simulink model "pmsm"  (R2025a)
settings: Solver=FixedStepAuto  StartTime=0.0  StopTime=5  RelTol=1e-3
model workspace (MAT data in the model file):
  pmsm_Ts = Simulink.Parameter
  pmsm_Ts.Value = 1e-05
  pmsm_Ts.Complexity = 'real'
  pmsm_Ts.Dimensions = [1 1]
  pmsm_Ts.DataType = 'auto'
  pmsm_Ts.DocUnits = 's'
  pmsm_Vcc = Simulink.Parameter
  pmsm_Vcc.Value = 40
  pmsm_Vcc.Complexity = 'real'
  pmsm_Vcc.Dimensions = [1 1]
  pmsm_Vcc.DataType = 'auto'
  pmsm_Vcc.DocUnits = 'V'
  pole_pairs = Simulink.Parameter
  pole_pairs.Value = 7
  pole_pairs.Complexity = 'real'
  pole_pairs.Dimensions = [1 1]
  pole_pairs.DataType = 'auto'
libraries: nesl_utility x5, fl_lib x4, ee_lib x3, simulink_extras x3, sdl_lib x1
settings Model: Creator=ascalzo  LastModifiedBy=mfussi
settings SolverCC: EnableFixedStepZeroCrossing=on
settings DataIOCC: SaveOutput=off  DSMLogging=off  SaveTime=off
settings DebuggingCC: ParameterPrecisionLossMsg=none  UnconnectedInputMsg=warning  UnconnectedOutputMsg=warning  UnconnectedLineMsg=warning
settings ModelReferenceCC: EnableRefExpFcnMdlSchedulingChecks=on
settings RTWCC: GPUComputeCapability=3.5  DLArmComputeVersion=19.05

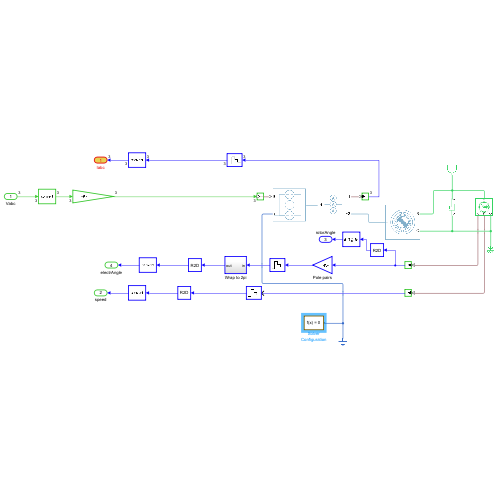
[thumbnail: Simulink's stored preview of the top-level diagram]
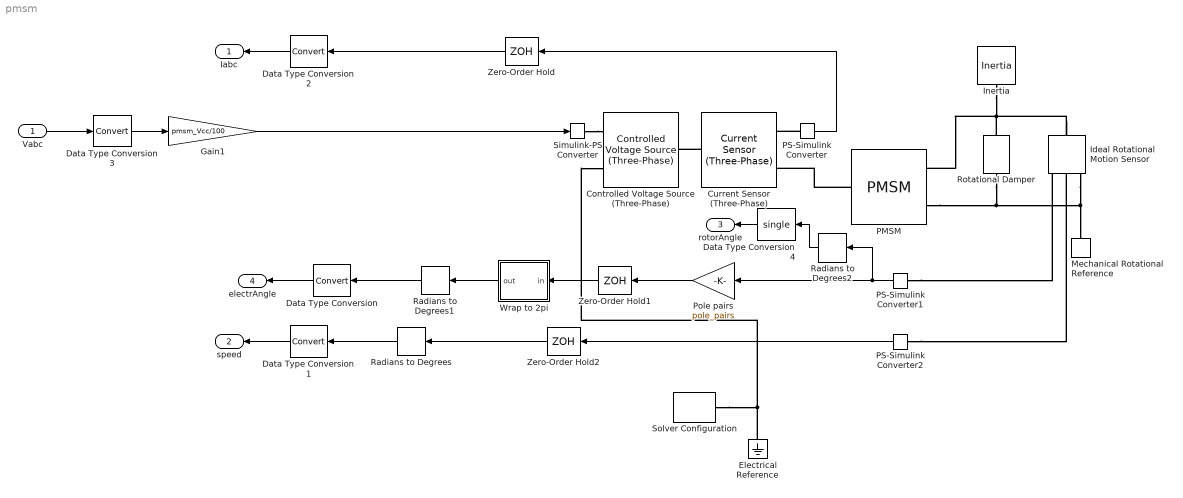
== system pmsm ==
  Vabc : Inport  OutDataTypeStr=single  Unit=%  PortDimensions=3  SampleTime=pmsm_Ts
  Controlled Voltage Source (Three-Phase) : ee_lib/Sources/Controlled Voltage Source (Three-Phase)  input_option=ee.enum.inputType.instantaneous  FRated=60 Hz
      settings: InternalSimscapePortConfiguration="{\"Bottom\":[],\"Left\":[{\"id\":\"S\",\"label\":\"S\",\"type\":\"input\"},{\"id\":\"n\",\"label\":\"n\",\"type\":\"foundation.electrical.electrical\"}],\"Right\":[{\"id\":\"N\",\"label\":\"~\",\"type\":\"foundation.electrical.three_phase\"}],\"Top\":[]}"
  Current Sensor (Three-Phase) : ee_lib/Sensors & Transducers/Current Sensor (Three-Phase)
  Data Type Conversion{,1..3} (4 alike) : DataTypeConversion  SaturateOnIntegerOverflow=off  RndMeth=Floor
  Data Type Conversion4 : DataTypeConversion  OutDataTypeStr=single  SaturateOnIntegerOverflow=off  RndMeth=Floor
  Electrical Reference : fl_lib/Electrical/Electrical Elements/Electrical Reference
  Gain1 : Gain  Gain=pmsm_Vcc/100
  Ideal Rotational Motion Sensor : fl_lib/Mechanical/Mechanical Sensors/Ideal Rotational Motion Sensor  reference=foundation.enum.MeasurementReference.difference  acceleration_port=false  velocity_port=true  position_port=true  wrap_angle=false  offset=0 rad
  Inertia : fl_lib/Mechanical/Rotational Elements/Inertia  inertia=3 g*cm^2  num_ports=foundation.enum.numPorts2.one  w_specify=off  w_priority=High  w=0 rad/s  w_nominal_specify=off  w_nominal_value=1  w_nominal_unit=rad/s  t_specify=off  t_priority=None  t=0 N*m  t_nominal_specify=off  t_nominal_value=1  t_nominal_unit=N*m
  Mechanical Rotational Reference : fl_lib/Mechanical/Rotational Elements/Mechanical Rotational Reference
  PMSM : ee_lib/Electromechanical/Permanent Magnet/PMSM  port_option=ee.enum.threePhasePort.composite  winding_type=ee.enum.statorconnection.wye  machine_param=ee.enum.pmsm.parameterization.constant  nPolePairs=pole_pairs  pmflux_param=ee.enum.pmflux.torqueconstant  pm_flux_linkage=0.03 Wb  torque_constant=32.2*2/3 mN*m/A  back_emf_constant=0.18 V/(rad/s)  stator_param=ee.enum.statorparam.LsLmMs  Ld=0.00019 H  Lq=0.00025 H  idVec=[-200, 0, 200] A  iqVec=[-200, 0, 200] A  LdMatrix=0.0002 * ones(3, 3) H  LqMatrix=0.0002 * ones(3, 3) H  PmMatrix=0.1 * ones(3, 3) Wb  ktMatrix=0.18 * ones(3, 3) N*m/A  keMatrix=0.18 * ones(3, 3) V/(rad/s)  L0=0.00016 H  Ls=3150/3 uH  Lm=-0.1*3150/3*0 uH  Ms=(3150/3)/2 uH  Rs=0.9 % 25.9/2 Ohm  zero_sequence=ee.enum.park.zerosequence.exclude  axes_param=ee.enum.rotorangle.daxis  loss_param=ee.enum.ironloss.none  losses_oc=[0, 0, 0] W  losses_sc=[0, 0, 0] W  f_losses=60 Hz  Isc_losses=95 A  J=3.3 g*cm^2  lam=7.4e-5 m*mN/rpm  i_d_specify=off  i_d_priority=None  i_d=0 A  i_d_nominal_specify=off  i_d_nominal_value=1  i_d_nominal_unit=A  i_q_specify=off  i_q_priority=None  i_q=0 A  i_q_nominal_specify=off  i_q_nominal_value=1  i_q_nominal_unit=A  torque_specify=off  torque_priority=None  torque=0 N*m  torque_nominal_specify=off  torque_nominal_value=1  torque_nominal_unit=N*m  angular_velocity_specify=on  angular_velocity_priority=High  angular_velocity=0 rpm  angular_velocity_nominal_specify=off  angular_velocity_nominal_value=1  angular_velocity_nominal_unit=rpm  angular_position_specify=on  angular_position_priority=High  angular_position=0 deg  angular_position_nominal_specify=off  angular_position_nominal_value=1  angular_position_nominal_unit=deg  alpha=3.93e-3 1/K  alpha_flux=-0.001 1/K  Tmeas=298.15 K  stator_thermal_mass=100 J/K  rotor_thermal_mass=200 J/K  Rm_percent_rotor=90  Rd_percent_rotor=30  temperatureA_specify=off  temperatureA_priority=High  temperatureA=25 degC  temperatureA_nominal_specify=off  temperatureA_nominal_value=1  temperatureA_nominal_unit=degC  temperatureB_specify=off  temperatureB_priority=High  temperatureB=25 degC  temperatureB_nominal_specify=off  temperatureB_nominal_value=1  temperatureB_nominal_unit=degC  temperatureC_specify=off  temperatureC_priority=High  temperatureC=25 degC  temperatureC_nominal_specify=off  temperatureC_nominal_value=1  temperatureC_nominal_unit=degC  temperatureR_specify=off  temperatureR_priority=High  temperatureR=25 degC  temperatureR_nominal_specify=off  temperatureR_nominal_value=1  temperatureR_nominal_unit=degC
      settings: InternalSimscapePortConfiguration="{\"Bottom\":[],\"Left\":[{\"id\":\"N\",\"label\":\"~\",\"type\":\"foundation.electrical.three_phase\"}],\"Right\":[{\"id\":\"R\",\"label\":\"R\",\"type\":\"foundation.mechanical.rotational.rotational\"},{\"id\":\"C\",\"label\":\"C\",\"type\":\"foundation.mechanical.rotational.rotational\"}],\"Top\":[]}"
  PS-Simulink Converter : nesl_utility/PS-Simulink Converter  PhysicalDomain=network_engine_domain  SubClassName=ps_output  LeftPortType=input  RightPortType=output  PseudoPeriodic=off  Frequencies=[]  VectorFormat=1-D array  Unit=A  AffineConversion=off
  PS-Simulink Converter1 : nesl_utility/PS-Simulink Converter  PhysicalDomain=network_engine_domain  SubClassName=ps_output  LeftPortType=input  RightPortType=output  PseudoPeriodic=off  Frequencies=[]  VectorFormat=1-D array  Unit=rad  AffineConversion=off
  PS-Simulink Converter2 : nesl_utility/PS-Simulink Converter  PhysicalDomain=network_engine_domain  SubClassName=ps_output  LeftPortType=input  RightPortType=output  PseudoPeriodic=off  Frequencies=[]  VectorFormat=1-D array  Unit=inherit  AffineConversion=off
  Pole pairs : Gain  Gain=pole_pairs
  Radians to Degrees : simulink_extras/Transformations/Radians to Degrees
  Radians to Degrees1 : simulink_extras/Transformations/Radians to Degrees
  Radians to Degrees2 : simulink_extras/Transformations/Radians to Degrees
  Rotational Damper : sdl_lib/Couplings & Drives/Springs & Dampers/Rotational Damper  D=7.45e-3 m*mN/rpm  thermal_port=simscape.enum.thermaleffects.omit  thermal_mass=50 kJ/K  temperature_specify=off  temperature_priority=High  temperature=300 K  temperature_nominal_specify=off  temperature_nominal_value=1  temperature_nominal_unit=K
  Simulink-PS Converter : nesl_utility/Simulink-PS Converter  PhysicalDomain=network_engine_domain  SubClassName=ps_input  LeftPortType=input  RightPortType=output  PseudoPeriodic=off  Frequencies=[]  NoiseDistribution=none  NoiseParameters=[]  Unit=V  AffineConversion=off  FilteringAndDerivatives=provide  SimscapeFilterOrder=1  InputFilterTimeConstant=0.001  UdotUserProvided=0
  Solver Configuration : nesl_utility/Solver Configuration  PhysicalDomain=network_engine_domain  SubClassName=solver  LeftPortType=input  RightPortType=generic  Tones=[]  Harmonics=[]  SimulateNoise=off  Profile=off  UseLocalSampling=off  EnableSwitchedLinearOptims=on  FrequencyDomain=off  UseCCode=off  RelTol=0.001  AbsTol=1e-06  MinStep=1e-09  ToWorkspace=off  RevertToSquareIcSolve=off  NumHomotopyIterations=100  PhasorMode=off  PhasorModeNumHarmonics=1  ConsistencySolver=NEWTON_XTOL_AFTER_FTOL  IndexReductionMethod=DerivativeReplacement  DoDC=off  ResidualTolerance=1e-09  ConsistencyTolSource=GLOBAL  ConsistencyAbsTol=0.001  ConsistencyRelTol=0.001  ConsistencyTolFactor=0.001  UseLocalSolver=on  LocalSolverChoice=NE_BACKWARD_EULER_ADVANCER  ResolveIndetEquations=on  FunctionEvalNumThread=1  LocalSolverSampleTime=pmsm_Ts  DoFixedCost=on  MaxNonlinIter=3  MaxModeIter=2  ComputeImpulses=on  ImpulseIterations=2  LinearAlgebra=auto  LinearAlgebraNumThread=0  EquationFormulation=NE_TIME_EF  DelaysMemoryBudget=1024  AutomaticFiltering=on  FilteringTimeConstant=1e-6  PartitionStorageMethod=AS_NEEDED  PartitionMemoryBudget=1024  PartitionMethod=ROBUST  MultibodyUseLocalSolver=off  MultibodyLocalSolverChoice=ODE1  MultibodyLocalSolverSampleTime=0.001
  Wrap to 2pi : Subsystem
  Zero-Order Hold : ZeroOrderHold  SampleTime=-1
  Zero-Order Hold1 : ZeroOrderHold  SampleTime=-1
  Zero-Order Hold2 : ZeroOrderHold  SampleTime=-1
  Iabc : Outport  OutDataTypeStr=single  Unit=A  PortDimensions=3  SampleTime=pmsm_Ts
  speed : Outport  Port=2  OutDataTypeStr=single  Unit=deg/s  PortDimensions=1  SampleTime=pmsm_Ts
  rotorAngle : Outport  Port=3
  electrAngle : Outport  Port=4  OutDataTypeStr=single  Unit=deg  PortDimensions=1  SampleTime=pmsm_Ts
  wires:
  PS-Simulink Converter2/1 -> Zero-Order Hold2/1
  PS-Simulink Converter/1 -> Zero-Order Hold/1
  Zero-Order Hold/1 -> Data Type Conversion2/1
  Radians to Degrees/1 -> Data Type Conversion1/1
  Zero-Order Hold2/1 -> Radians to Degrees/1
  Data Type Conversion2/1 -> Iabc/1
  Pole pairs/1 -> Zero-Order Hold1/1
  Data Type Conversion/1 -> electrAngle/1
  Vabc/1 -> Data Type Conversion3/1
  Data Type Conversion3/1 -> Gain1/1
  Data Type Conversion1/1 -> speed/1
  Gain1/1 -> Simulink-PS Converter/1
  Radians to Degrees1/1 -> Data Type Conversion/1
  Zero-Order Hold1/1 -> Wrap to 2pi/1(in)
  Wrap to 2pi/1(out) -> Radians to Degrees1/1
  PS-Simulink Converter1/1 -> Pole pairs/1, Radians to Degrees2/1
  Data Type Conversion4/1 -> rotorAngle/1
  Radians to Degrees2/1 -> Data Type Conversion4/1
  connections:
  Solver Configuration/RConn1 -- Controlled Voltage Source (Three-Phase)/LConn2 -- Electrical Reference/LConn1
  Inertia/LConn1 -- Ideal Rotational Motion Sensor/LConn1 -- PMSM/RConn1 -- Rotational Damper/LConn1
  PMSM/RConn2 -- Rotational Damper/RConn1 -- Ideal Rotational Motion Sensor/RConn1 -- Mechanical Rotational Reference/LConn1
  Current Sensor (Three-Phase)/LConn1 -- Controlled Voltage Source (Three-Phase)/RConn1
  PS-Simulink Converter2/LConn1 -- Ideal Rotational Motion Sensor/RConn2
  PS-Simulink Converter/LConn1 -- Current Sensor (Three-Phase)/RConn1
  PMSM/LConn1 -- Current Sensor (Three-Phase)/RConn2
  Simulink-PS Converter/RConn1 -- Controlled Voltage Source (Three-Phase)/LConn1
  PS-Simulink Converter1/LConn1 -- Ideal Rotational Motion Sensor/RConn3

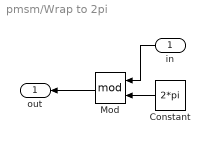
== system pmsm/Wrap to 2pi ==
  in : Inport
  Constant : Constant  Value=2*pi
  Mod : Math  Operator=mod  OutputSignalType=real
  out : Outport
  wires:
  Constant/1 -> Mod/2
  Mod/1 -> out/1
  in/1 -> Mod/1
